simulink model "VehiclePlant"  (R2026b)
settings: Solver=VariableStepAuto  StopTime=60
undefined symbols (not defined in the file): Drag, VehicleMass
settings Model: DataDictionary=CruiseControlData.sldd  Creator=christopher  LastModifiedBy=christopher

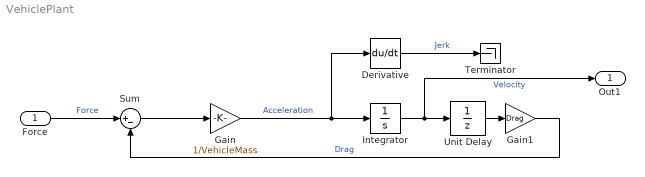
== system VehiclePlant ==
  Force : Inport
  Derivative : Derivative
  Gain : Gain  Gain=1/VehicleMass
  Gain1 : Gain  Gain=Drag
  Integrator : Integrator
  Sum : Sum  Inputs=|+-
  Terminator : Terminator
  Unit Delay : UnitDelay  SampleTime=-1
  Out1 : Outport
  wires:
  Force/1 -> Sum/1  "Force"
  Sum/1 -> Gain/1
  Gain/1 -> Derivative/1, Integrator/1  "Acceleration"
  Derivative/1 -> Terminator/1  "Jerk"
  Gain1/1 -> Sum/2  "Drag"
  Unit Delay/1 -> Gain1/1
  Integrator/1 -> Out1/1, Unit Delay/1  "Velocity"
